simulink model "task2_firm_Shapovalov"  (R2023a)
settings: Solver=ode45  StartTime=0  StopTime=200  RelTol=1e-6  AbsTol=1e-9
InitFcn:
  | alpha=5; beta=8; delta=1; mu=2.1; sigma=4.1; gamma=1; x0=1; y0=1; z0=1;
Description:
  | Zadanie 2 (2.25): x-kredit, y-kapital, z-chislennost. Menyayte gamma v [0;10].
settings Model: Creator=maybn  LastModifiedBy=maybn
settings OptimizationCC: BlockReduction=off  BooleanDataType=off
settings DebuggingCC: SaveWithParameterizedLinksMsg=none  UnderspecifiedInitializationDetection=Classic  MergeDetectMultiDrivingBlocksExec=none  SignalResolutionControl=TryResolveAllWithWarning
settings HardwareCC: TargetUnknown=on
settings ModelReferenceCC: PropagateSignalLabelsOutOfModel=off

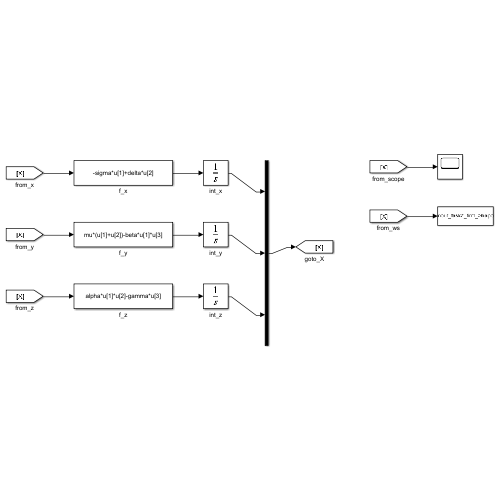
[thumbnail: Simulink's stored preview of the top-level diagram]
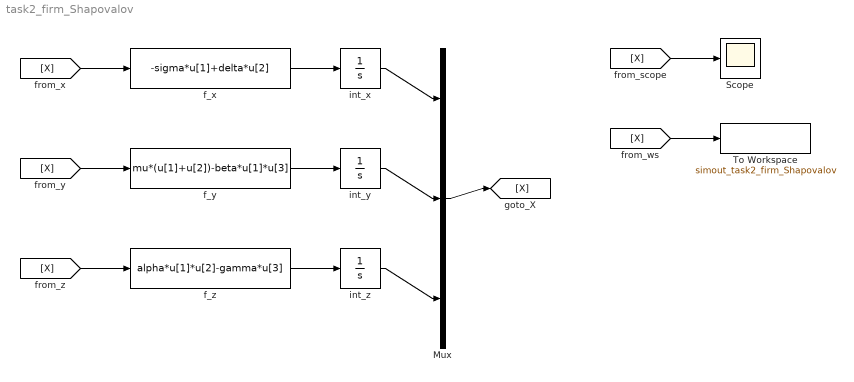
== system task2_firm_Shapovalov ==
  Mux : Mux  Inputs=3
  Scope : Scope
  To Workspace : ToWorkspace  VariableName=simout_task2_firm_Shapovalov
  f_x : Fcn  Expr=-sigma*u[1]+delta*u[2]
  f_y : Fcn  Expr=mu*(u[1]+u[2])-beta*u[1]*u[3]
  f_z : Fcn  Expr=alpha*u[1]*u[2]-gamma*u[3]
  int_x : Integrator  InitialCondition=x0
  int_y : Integrator  InitialCondition=y0
  int_z : Integrator  InitialCondition=z0
  wires:
  [X] -> f_x/1
  f_x/1 -> int_x/1
  int_x/1 -> Mux/1
  [X] -> f_y/1
  f_y/1 -> int_y/1
  int_y/1 -> Mux/2
  [X] -> f_z/1
  f_z/1 -> int_z/1
  int_z/1 -> Mux/3
  Mux/1 -> [X]
  [X] -> Scope/1
  [X] -> To Workspace/1
